simulink model "pot_led_suave"  (R2026b)
settings: Solver=FixedStepDiscrete  StopTime=1  FixedStep=0.01  EnableMultiTasking=on
libraries: arduinolib x2
settings Model: SILPILModeSetting=veronly  Creator=dlynchr  LastModifiedBy=dlynchr
settings SolverCC: AutoInsertRateTranBlk=on
settings OptimizationCC: DifferentSizesBufferReuse=on  EfficientTunableParamExpr=on  EnhancedBackFolding=on  MaxStackSize=64  OptimizationCustomize=off  OptimizeBlockOrder=speed  PassReuseOutputArgsAs=Individual arguments  RemoveInternalMemoryZeroInit=on  RemoveRootLevelIOMemoryZeroInit=on
settings DebuggingCC: ParameterTunabilityLossMsg=error
settings HardwareCC: ProdHWDeviceType=Atmel->AVR  ProdLargestAtomicFloat=None
settings SFSimCC: MATLABDynamicMemAlloc=off
settings RTWCC: BuildConfiguration=Faster Runs  Description=Embedded Coder  GenerateReport=on  HardwareBoard=Arduino Uno  SystemTargetFile=ert.tlc  TLCOptions=-aInlineSetEventsForThisBaseRateFcn=TLC_FALSE -aSuppressMultiTaskScheduler=TLC_FALSE -aRateBasedStepFcn=1  TemplateMakefile=ert_default_tmf  Toolchain=Arduino AVR
settings CodeAppCC: ForceParamTrailComments=on  IgnoreCustomStorageClasses=off  InsertBlockDesc=on  OperatorAnnotations=on  SFDataObjDesc=on  SimulinkDataObjDesc=on
settings ERTTargetCC: CombineSignalStateStructs=on  ExtModeAutomaticAllocSize=off  ExtModeIntrfLevel=Level2 - Open  ExtModeMexFile=ext_xcp  ExtModeStaticAlloc=on  SupportContinuousTime=on  SupportVariableSizeSignals=on

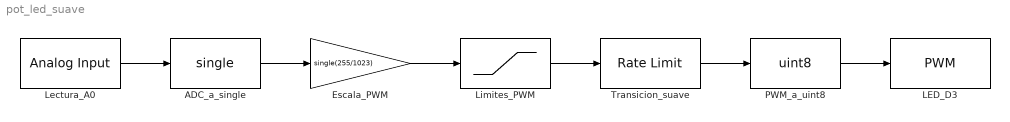
== system pot_led_suave ==
  ADC_a_single : DataTypeConversion  OutDataTypeStr=single  SaturateOnIntegerOverflow=off  RndMeth=Floor
  Escala_PWM : Gain  Gain=single(255/1023)  OutDataTypeStr=single
  LED_D3 : arduinolib/PWM  pinNumber=3  frequencyType=Default  desiredFrequency=490.2  achievableFrequency=490.2
  Lectura_A0 : arduinolib/Analog Input  pinNumber=0  ReadResultsOnly=off  ConversionTriggerSource=Software  ExternalTriggerType=uint32( 0 )  OutputDataType=uint16  EnableConversionCompleteNotify=off  EnableOuputStatus=off  SampleTime=0.01  blockPlatform=arduino
  Limites_PWM : Saturate  UpperLimit=255  LowerLimit=0
  PWM_a_uint8 : DataTypeConversion  OutDataTypeStr=uint8  RndMeth=Floor
  Transicion_suave : RateLimiter  RisingSlewLimit=single(100)  FallingSlewLimit=single(-100)  SampleTimeMode=inherited  InitialCondition=single(0)
  wires:
  Lectura_A0/1 -> ADC_a_single/1
  ADC_a_single/1 -> Escala_PWM/1
  Escala_PWM/1 -> Limites_PWM/1
  PWM_a_uint8/1 -> LED_D3/1
  Limites_PWM/1 -> Transicion_suave/1
  Transicion_suave/1 -> PWM_a_uint8/1
